simulink model "RRTMS_System_Architecture"  (R2026a)
settings: Solver=VariableStepAuto
settings Model: Creator=HP  LastModifiedBy=HP

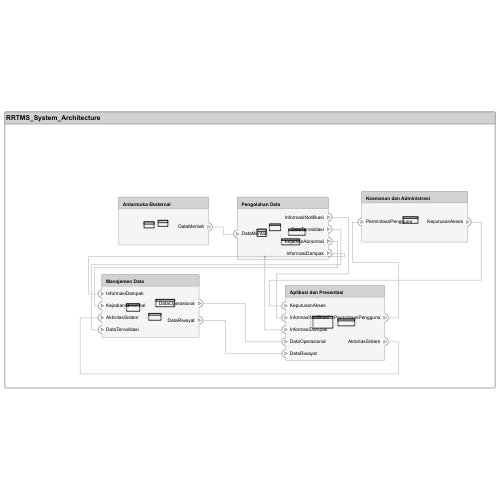
[thumbnail: Simulink's stored preview of the top-level diagram]
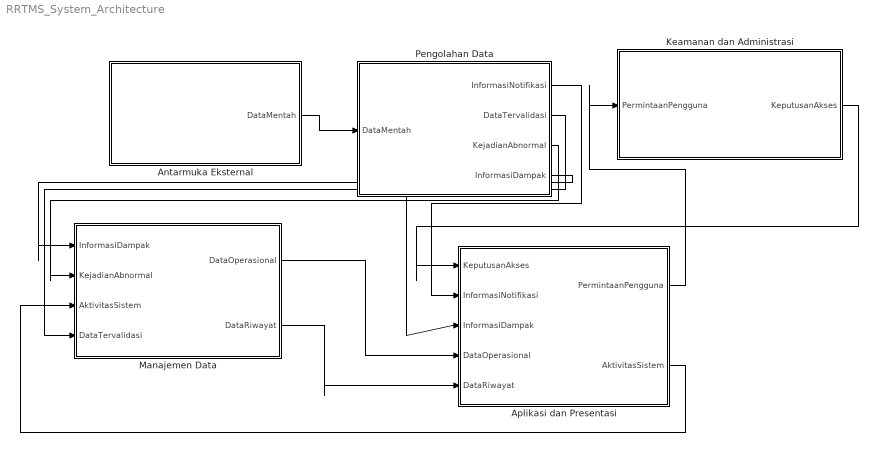
== system RRTMS_System_Architecture ==
  Antarmuka Eksternal : Subsystem
      settings: PortSchema="{\"entries\":[{\"content\":{\"headerSize\":26,\"margin\":15,\"minimumSpacing\":25,\"sides\":[{\"content\":{},\"type\":\"ConnectorPlacement.EquallySpacedRectSide\",\"uuid\":\"71f00674-931b-470b-b0fd-a692bb3b3063\"},{\"content\":{\"connectorIds\":[\"Out1\"],\"side\":\"RIGHT\"},\"type\":\"ConnectorPlacement.EquallySpacedRectSide\",\"uuid\":\"86d6e0cc-71b2-4a9b-97f1-d24c94197c14\"},{\"content\":{\"side\":\"TOP\"},\"type\":\"ConnectorPlacement.EquallySpacedRectSide\",\"uuid\":\"2847748d-1182-42d4-93ed-9e0e7089bed0\"}]},\"type\":\"ConnectorPlacement.EquallySpacedConnector\",\"uuid\":\"b969c393-021a-4397-a00e-d7d17b1fb0f6\"}],\"packageUris\":[\"http://schema.mathworks.com/mf0/Connector/R2020b\"],\"version\":\"1.0\"}"
  Aplikasi dan Presentasi : Subsystem
      settings: PortSchema="{\"entries\":[{\"content\":{\"headerSize\":26,\"margin\":15,\"minimumSpacing\":25,\"sides\":[{\"content\":{\"connectorIds\":[\"In1\",\"In2\",\"In5\",\"In3\",\"In4\"]},\"type\":\"ConnectorPlacement.EquallySpacedRectSide\",\"uuid\":\"71f00674-931b-470b-b0fd-a692bb3b3063\"},{\"content\":{\"connectorIds\":[\"Out1\",\"Out2\"],\"side\":\"RIGHT\"},\"type\":\"ConnectorPlacement.EquallySpacedRectSide\",\"uuid\":\"86d6e0cc-71b2-4a9b-97f1-d24c94197c14\"},{\"content\":{\"side\":\"TOP\"},\"type\":\"ConnectorPlacement.EquallySpacedRectSide\",\"uuid\":\"2847748d-1182-42d4-93ed-9e0e7089bed0\"}]},\"type\":\"ConnectorPlacement.EquallySpacedConnector\",\"uuid\":\"b969c393-021a-4397-a00e-d7d17b1fb0f6\"}],\"packageUris\":[\"http://schema.mathworks.com/mf0/Connector/R2020b\"],\"version\":\"1.0\"}"
  Keamanan dan Administrasi : Subsystem
      settings: PortSchema="{\"entries\":[{\"content\":{\"headerSize\":26,\"margin\":15,\"minimumSpacing\":25,\"sides\":[{\"content\":{\"connectorIds\":[\"In1\"]},\"type\":\"ConnectorPlacement.EquallySpacedRectSide\",\"uuid\":\"71f00674-931b-470b-b0fd-a692bb3b3063\"},{\"content\":{\"connectorIds\":[\"Out1\"],\"side\":\"RIGHT\"},\"type\":\"ConnectorPlacement.EquallySpacedRectSide\",\"uuid\":\"86d6e0cc-71b2-4a9b-97f1-d24c94197c14\"},{\"content\":{\"side\":\"TOP\"},\"type\":\"ConnectorPlacement.EquallySpacedRectSide\",\"uuid\":\"2847748d-1182-42d4-93ed-9e0e7089bed0\"}]},\"type\":\"ConnectorPlacement.EquallySpacedConnector\",\"uuid\":\"b969c393-021a-4397-a00e-d7d17b1fb0f6\"}],\"packageUris\":[\"http://schema.mathworks.com/mf0/Connector/R2020b\"],\"version\":\"1.0\"}"
  Manajemen Data : Subsystem
      settings: PortSchema="{\"entries\":[{\"content\":{\"headerSize\":26,\"margin\":15,\"minimumSpacing\":25,\"sides\":[{\"content\":{\"connectorIds\":[\"In1\",\"In2\",\"In3\",\"In4\"]},\"type\":\"ConnectorPlacement.EquallySpacedRectSide\",\"uuid\":\"71f00674-931b-470b-b0fd-a692bb3b3063\"},{\"content\":{\"connectorIds\":[\"Out2\",\"Out1\"],\"side\":\"RIGHT\"},\"type\":\"ConnectorPlacement.EquallySpacedRectSide\",\"uuid\":\"86d6e0cc-71b2-4a9b-97f1-d24c94197c14\"},{\"content\":{\"side\":\"TOP\"},\"type\":\"ConnectorPlacement.EquallySpacedRectSide\",\"uuid\":\"2847748d-1182-42d4-93ed-9e0e7089bed0\"}]},\"type\":\"ConnectorPlacement.EquallySpacedConnector\",\"uuid\":\"b969c393-021a-4397-a00e-d7d17b1fb0f6\"}],\"packageUris\":[\"http://schema.mathworks.com/mf0/Connector/R2020b\"],\"version\":\"1.0\"}"
  Pengolahan Data : Subsystem
      settings: PortSchema="{\"entries\":[{\"content\":{\"headerSize\":26,\"margin\":15,\"minimumSpacing\":25,\"sides\":[{\"content\":{\"connectorIds\":[\"In1\"]},\"type\":\"ConnectorPlacement.EquallySpacedRectSide\",\"uuid\":\"71f00674-931b-470b-b0fd-a692bb3b3063\"},{\"content\":{\"connectorIds\":[\"Out1\",\"Out3\",\"Out4\",\"Out2\"],\"side\":\"RIGHT\"},\"type\":\"ConnectorPlacement.EquallySpacedRectSide\",\"uuid\":\"86d6e0cc-71b2-4a9b-97f1-d24c94197c14\"},{\"content\":{\"side\":\"TOP\"},\"type\":\"ConnectorPlacement.EquallySpacedRectSide\",\"uuid\":\"2847748d-1182-42d4-93ed-9e0e7089bed0\"}]},\"type\":\"ConnectorPlacement.EquallySpacedConnector\",\"uuid\":\"b969c393-021a-4397-a00e-d7d17b1fb0f6\"}],\"packageUris\":[\"http://schema.mathworks.com/mf0/Connector/R2020b\"],\"version\":\"1.0\"}"
  wires:
  Antarmuka Eksternal/1(DataMentah) -> Pengolahan Data/1(DataMentah)
  Pengolahan Data/3(DataTervalidasi) -> Manajemen Data/4(DataTervalidasi)
  Pengolahan Data/4(KejadianAbnormal) -> Manajemen Data/2(KejadianAbnormal)
  Pengolahan Data/2(InformasiDampak) -> Aplikasi dan Presentasi/5(InformasiDampak), Manajemen Data/1(InformasiDampak)
  Manajemen Data/2(DataOperasional) -> Aplikasi dan Presentasi/3(DataOperasional)
  Manajemen Data/1(DataRiwayat) -> Aplikasi dan Presentasi/4(DataRiwayat)
  Pengolahan Data/1(InformasiNotifikasi) -> Aplikasi dan Presentasi/2(InformasiNotifikasi)
  Aplikasi dan Presentasi/2(AktivitasSistem) -> Manajemen Data/3(AktivitasSistem)
  Aplikasi dan Presentasi/1(PermintaanPengguna) -> Keamanan dan Administrasi/1(PermintaanPengguna)
  Keamanan dan Administrasi/1(KeputusanAkses) -> Aplikasi dan Presentasi/1(KeputusanAkses)

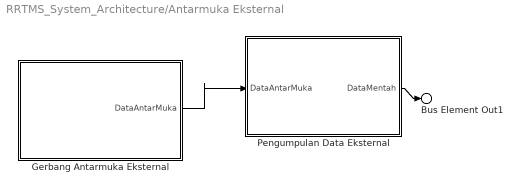
== system RRTMS_System_Architecture/Antarmuka Eksternal ==
  Gerbang Antarmuka Eksternal : Subsystem
      settings: PortSchema="{\"entries\":[{\"content\":{\"headerSize\":26,\"margin\":15,\"minimumSpacing\":25,\"sides\":[{\"content\":{},\"type\":\"ConnectorPlacement.EquallySpacedRectSide\",\"uuid\":\"71f00674-931b-470b-b0fd-a692bb3b3063\"},{\"content\":{\"connectorIds\":[\"Out1\"],\"side\":\"RIGHT\"},\"type\":\"ConnectorPlacement.EquallySpacedRectSide\",\"uuid\":\"86d6e0cc-71b2-4a9b-97f1-d24c94197c14\"},{\"content\":{\"side\":\"TOP\"},\"type\":\"ConnectorPlacement.EquallySpacedRectSide\",\"uuid\":\"2847748d-1182-42d4-93ed-9e0e7089bed0\"}]},\"type\":\"ConnectorPlacement.EquallySpacedConnector\",\"uuid\":\"b969c393-021a-4397-a00e-d7d17b1fb0f6\"}],\"packageUris\":[\"http://schema.mathworks.com/mf0/Connector/R2020b\"],\"version\":\"1.0\"}"
  Pengumpulan Data Eksternal : Subsystem
      settings: PortSchema="{\"entries\":[{\"content\":{\"headerSize\":26,\"margin\":15,\"minimumSpacing\":25,\"sides\":[{\"content\":{\"connectorIds\":[\"In1\"]},\"type\":\"ConnectorPlacement.EquallySpacedRectSide\",\"uuid\":\"71f00674-931b-470b-b0fd-a692bb3b3063\"},{\"content\":{\"connectorIds\":[\"Out1\"],\"side\":\"RIGHT\"},\"type\":\"ConnectorPlacement.EquallySpacedRectSide\",\"uuid\":\"86d6e0cc-71b2-4a9b-97f1-d24c94197c14\"},{\"content\":{\"side\":\"TOP\"},\"type\":\"ConnectorPlacement.EquallySpacedRectSide\",\"uuid\":\"2847748d-1182-42d4-93ed-9e0e7089bed0\"}]},\"type\":\"ConnectorPlacement.EquallySpacedConnector\",\"uuid\":\"b969c393-021a-4397-a00e-d7d17b1fb0f6\"}],\"packageUris\":[\"http://schema.mathworks.com/mf0/Connector/R2020b\"],\"version\":\"1.0\"}"
  Bus Element Out1 : Outport  PortName=DataMentah
  wires:
  Gerbang Antarmuka Eksternal/1(DataAntarMuka) -> Pengumpulan Data Eksternal/1(DataAntarMuka)
  Pengumpulan Data Eksternal/1(DataMentah) -> Bus Element Out1/1

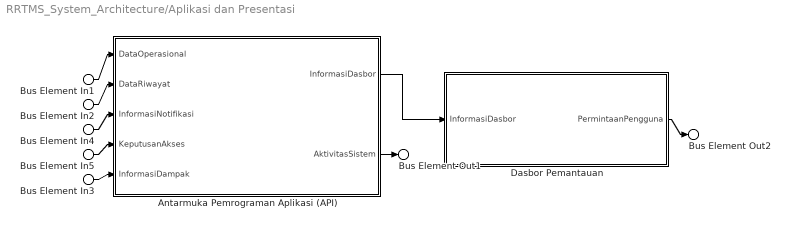
== system RRTMS_System_Architecture/Aplikasi dan Presentasi ==
  Bus Element In5 : Inport  PortName=KeputusanAkses
  Bus Element In4 : Inport  Port=2  PortName=InformasiNotifikasi
  Bus Element In1 : Inport  Port=3  PortName=DataOperasional
  Bus Element In2 : Inport  Port=4  PortName=DataRiwayat
  Bus Element In3 : Inport  Port=5  PortName=InformasiDampak
  Antarmuka Pemrograman Aplikasi (API) : Subsystem
      settings: PortSchema="{\"entries\":[{\"content\":{\"headerSize\":26,\"margin\":15,\"minimumSpacing\":25,\"sides\":[{\"content\":{\"connectorIds\":[\"In1\",\"In2\",\"In3\",\"In4\",\"In5\"]},\"type\":\"ConnectorPlacement.EquallySpacedRectSide\",\"uuid\":\"71f00674-931b-470b-b0fd-a692bb3b3063\"},{\"content\":{\"connectorIds\":[\"Out1\",\"Out2\"],\"side\":\"RIGHT\"},\"type\":\"ConnectorPlacement.EquallySpacedRectSide\",\"uuid\":\"86d6e0cc-71b2-4a9b-97f1-d24c94197c14\"},{\"content\":{\"side\":\"TOP\"},\"type\":\"ConnectorPlacement.EquallySpacedRectSide\",\"uuid\":\"2847748d-1182-42d4-93ed-9e0e7089bed0\"}]},\"type\":\"ConnectorPlacement.EquallySpacedConnector\",\"uuid\":\"b969c393-021a-4397-a00e-d7d17b1fb0f6\"}],\"packageUris\":[\"http://schema.mathworks.com/mf0/Connector/R2020b\"],\"version\":\"1.0\"}"
  Dasbor Pemantauan : Subsystem
      settings: PortSchema="{\"entries\":[{\"content\":{\"headerSize\":26,\"margin\":15,\"minimumSpacing\":25,\"sides\":[{\"content\":{\"connectorIds\":[\"In1\"]},\"type\":\"ConnectorPlacement.EquallySpacedRectSide\",\"uuid\":\"71f00674-931b-470b-b0fd-a692bb3b3063\"},{\"content\":{\"connectorIds\":[\"Out1\"],\"side\":\"RIGHT\"},\"type\":\"ConnectorPlacement.EquallySpacedRectSide\",\"uuid\":\"86d6e0cc-71b2-4a9b-97f1-d24c94197c14\"},{\"content\":{\"side\":\"TOP\"},\"type\":\"ConnectorPlacement.EquallySpacedRectSide\",\"uuid\":\"2847748d-1182-42d4-93ed-9e0e7089bed0\"}]},\"type\":\"ConnectorPlacement.EquallySpacedConnector\",\"uuid\":\"b969c393-021a-4397-a00e-d7d17b1fb0f6\"}],\"packageUris\":[\"http://schema.mathworks.com/mf0/Connector/R2020b\"],\"version\":\"1.0\"}"
  Bus Element Out2 : Outport  PortName=PermintaanPengguna
  Bus Element Out1 : Outport  Port=2  PortName=AktivitasSistem
  wires:
  Bus Element In1/1 -> Antarmuka Pemrograman Aplikasi (API)/1(DataOperasional)
  Bus Element In2/1 -> Antarmuka Pemrograman Aplikasi (API)/2(DataRiwayat)
  Bus Element In3/1 -> Antarmuka Pemrograman Aplikasi (API)/5(InformasiDampak)
  Bus Element In4/1 -> Antarmuka Pemrograman Aplikasi (API)/3(InformasiNotifikasi)
  Antarmuka Pemrograman Aplikasi (API)/1(InformasiDasbor) -> Dasbor Pemantauan/1(InformasiDasbor)
  Antarmuka Pemrograman Aplikasi (API)/2(AktivitasSistem) -> Bus Element Out1/1
  Dasbor Pemantauan/1(PermintaanPengguna) -> Bus Element Out2/1
  Bus Element In5/1 -> Antarmuka Pemrograman Aplikasi (API)/4(KeputusanAkses)

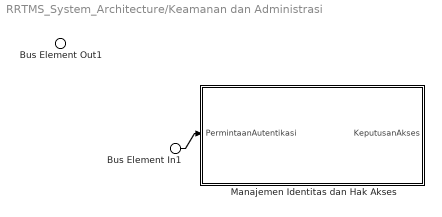
== system RRTMS_System_Architecture/Keamanan dan Administrasi ==
  Bus Element In1 : Inport  PortName=PermintaanPengguna
  Manajemen Identitas dan Hak Akses : Subsystem
      settings: PortSchema="{\"entries\":[{\"content\":{\"headerSize\":26,\"margin\":15,\"minimumSpacing\":25,\"sides\":[{\"content\":{\"connectorIds\":[\"In1\"]},\"type\":\"ConnectorPlacement.EquallySpacedRectSide\",\"uuid\":\"71f00674-931b-470b-b0fd-a692bb3b3063\"},{\"content\":{\"connectorIds\":[\"Out1\"],\"side\":\"RIGHT\"},\"type\":\"ConnectorPlacement.EquallySpacedRectSide\",\"uuid\":\"86d6e0cc-71b2-4a9b-97f1-d24c94197c14\"},{\"content\":{\"side\":\"TOP\"},\"type\":\"ConnectorPlacement.EquallySpacedRectSide\",\"uuid\":\"2847748d-1182-42d4-93ed-9e0e7089bed0\"}]},\"type\":\"ConnectorPlacement.EquallySpacedConnector\",\"uuid\":\"b969c393-021a-4397-a00e-d7d17b1fb0f6\"}],\"packageUris\":[\"http://schema.mathworks.com/mf0/Connector/R2020b\"],\"version\":\"1.0\"}"
  Bus Element Out1 : Outport  PortName=KeputusanAkses
  wires:
  Bus Element In1/1 -> Manajemen Identitas dan Hak Akses/1(PermintaanAutentikasi)

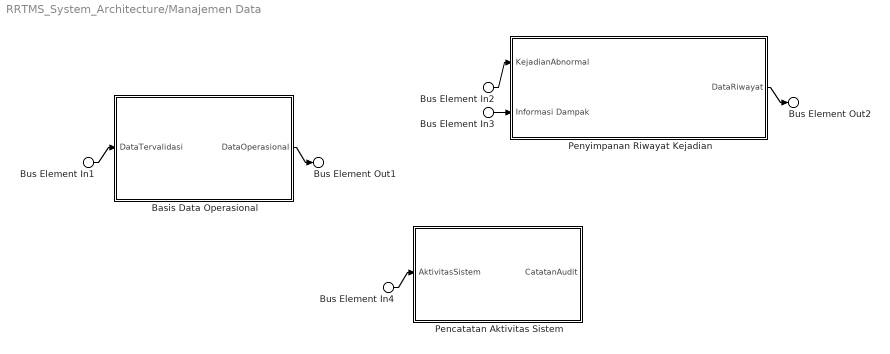
== system RRTMS_System_Architecture/Manajemen Data ==
  Bus Element In3 : Inport  PortName=InformasiDampak
  Bus Element In2 : Inport  Port=2  PortName=KejadianAbnormal
  Bus Element In4 : Inport  Port=3  PortName=AktivitasSistem
  Bus Element In1 : Inport  Port=4  PortName=DataTervalidasi
  Basis Data Operasional : Subsystem
      settings: PortSchema="{\"entries\":[{\"content\":{\"headerSize\":26,\"margin\":15,\"minimumSpacing\":25,\"sides\":[{\"content\":{\"connectorIds\":[\"In1\"]},\"type\":\"ConnectorPlacement.EquallySpacedRectSide\",\"uuid\":\"71f00674-931b-470b-b0fd-a692bb3b3063\"},{\"content\":{\"connectorIds\":[\"Out1\"],\"side\":\"RIGHT\"},\"type\":\"ConnectorPlacement.EquallySpacedRectSide\",\"uuid\":\"86d6e0cc-71b2-4a9b-97f1-d24c94197c14\"},{\"content\":{\"side\":\"TOP\"},\"type\":\"ConnectorPlacement.EquallySpacedRectSide\",\"uuid\":\"2847748d-1182-42d4-93ed-9e0e7089bed0\"}]},\"type\":\"ConnectorPlacement.EquallySpacedConnector\",\"uuid\":\"b969c393-021a-4397-a00e-d7d17b1fb0f6\"}],\"packageUris\":[\"http://schema.mathworks.com/mf0/Connector/R2020b\"],\"version\":\"1.0\"}"
  "Pencatatan Aktivitas Sistem " : Subsystem
      settings: PortSchema="{\"entries\":[{\"content\":{\"headerSize\":26,\"margin\":15,\"minimumSpacing\":25,\"sides\":[{\"content\":{\"connectorIds\":[\"In1\"]},\"type\":\"ConnectorPlacement.EquallySpacedRectSide\",\"uuid\":\"71f00674-931b-470b-b0fd-a692bb3b3063\"},{\"content\":{\"connectorIds\":[\"Out1\"],\"side\":\"RIGHT\"},\"type\":\"ConnectorPlacement.EquallySpacedRectSide\",\"uuid\":\"86d6e0cc-71b2-4a9b-97f1-d24c94197c14\"},{\"content\":{\"side\":\"TOP\"},\"type\":\"ConnectorPlacement.EquallySpacedRectSide\",\"uuid\":\"2847748d-1182-42d4-93ed-9e0e7089bed0\"}]},\"type\":\"ConnectorPlacement.EquallySpacedConnector\",\"uuid\":\"b969c393-021a-4397-a00e-d7d17b1fb0f6\"}],\"packageUris\":[\"http://schema.mathworks.com/mf0/Connector/R2020b\"],\"version\":\"1.0\"}"
  Penyimpanan Riwayat Kejadian : Subsystem
      settings: PortSchema="{\"entries\":[{\"content\":{\"headerSize\":26,\"margin\":15,\"minimumSpacing\":25,\"sides\":[{\"content\":{\"connectorIds\":[\"In1\",\"In2\"]},\"type\":\"ConnectorPlacement.EquallySpacedRectSide\",\"uuid\":\"71f00674-931b-470b-b0fd-a692bb3b3063\"},{\"content\":{\"connectorIds\":[\"Out1\"],\"side\":\"RIGHT\"},\"type\":\"ConnectorPlacement.EquallySpacedRectSide\",\"uuid\":\"86d6e0cc-71b2-4a9b-97f1-d24c94197c14\"},{\"content\":{\"side\":\"TOP\"},\"type\":\"ConnectorPlacement.EquallySpacedRectSide\",\"uuid\":\"2847748d-1182-42d4-93ed-9e0e7089bed0\"}]},\"type\":\"ConnectorPlacement.EquallySpacedConnector\",\"uuid\":\"b969c393-021a-4397-a00e-d7d17b1fb0f6\"}],\"packageUris\":[\"http://schema.mathworks.com/mf0/Connector/R2020b\"],\"version\":\"1.0\"}"
  Bus Element Out2 : Outport  PortName=DataRiwayat
  Bus Element Out1 : Outport  Port=2  PortName=DataOperasional
  wires:
  Bus Element In1/1 -> Basis Data Operasional/1(DataTervalidasi)
  Bus Element In2/1 -> Penyimpanan Riwayat Kejadian/1(KejadianAbnormal)
  Bus Element In3/1 -> Penyimpanan Riwayat Kejadian/2(Informasi Dampak)
  Basis Data Operasional/1(DataOperasional) -> Bus Element Out1/1
  Penyimpanan Riwayat Kejadian/1(DataRiwayat) -> Bus Element Out2/1
  Bus Element In4/1 -> "Pencatatan Aktivitas Sistem "/1(AktivitasSistem)

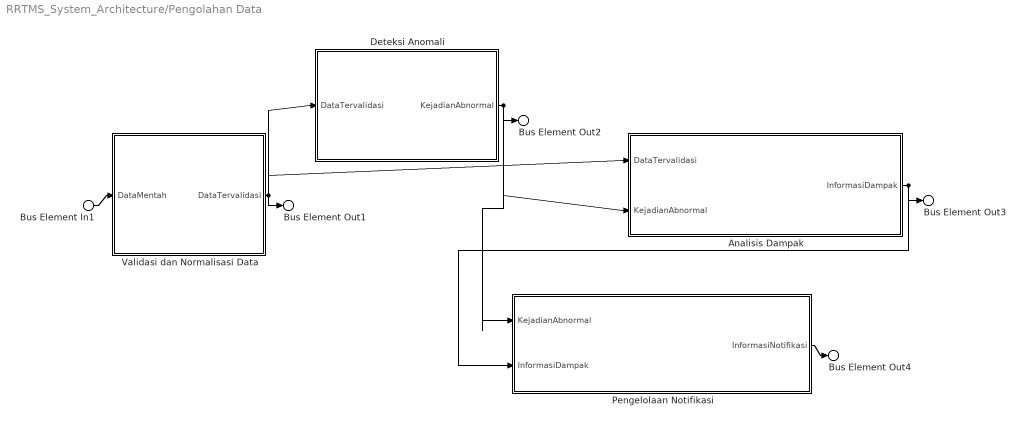
== system RRTMS_System_Architecture/Pengolahan Data ==
  Bus Element In1 : Inport  PortName=DataMentah
  Analisis Dampak : Subsystem
      settings: PortSchema="{\"entries\":[{\"content\":{\"headerSize\":26,\"margin\":15,\"minimumSpacing\":25,\"sides\":[{\"content\":{\"connectorIds\":[\"In1\",\"In2\"]},\"type\":\"ConnectorPlacement.EquallySpacedRectSide\",\"uuid\":\"71f00674-931b-470b-b0fd-a692bb3b3063\"},{\"content\":{\"connectorIds\":[\"Out1\"],\"side\":\"RIGHT\"},\"type\":\"ConnectorPlacement.EquallySpacedRectSide\",\"uuid\":\"86d6e0cc-71b2-4a9b-97f1-d24c94197c14\"},{\"content\":{\"side\":\"TOP\"},\"type\":\"ConnectorPlacement.EquallySpacedRectSide\",\"uuid\":\"2847748d-1182-42d4-93ed-9e0e7089bed0\"}]},\"type\":\"ConnectorPlacement.EquallySpacedConnector\",\"uuid\":\"b969c393-021a-4397-a00e-d7d17b1fb0f6\"}],\"packageUris\":[\"http://schema.mathworks.com/mf0/Connector/R2020b\"],\"version\":\"1.0\"}"
  Deteksi Anomali : Subsystem
      settings: PortSchema="{\"entries\":[{\"content\":{\"headerSize\":26,\"margin\":15,\"minimumSpacing\":25,\"sides\":[{\"content\":{\"connectorIds\":[\"In1\"]},\"type\":\"ConnectorPlacement.EquallySpacedRectSide\",\"uuid\":\"71f00674-931b-470b-b0fd-a692bb3b3063\"},{\"content\":{\"connectorIds\":[\"Out1\"],\"side\":\"RIGHT\"},\"type\":\"ConnectorPlacement.EquallySpacedRectSide\",\"uuid\":\"86d6e0cc-71b2-4a9b-97f1-d24c94197c14\"},{\"content\":{\"side\":\"TOP\"},\"type\":\"ConnectorPlacement.EquallySpacedRectSide\",\"uuid\":\"2847748d-1182-42d4-93ed-9e0e7089bed0\"}]},\"type\":\"ConnectorPlacement.EquallySpacedConnector\",\"uuid\":\"b969c393-021a-4397-a00e-d7d17b1fb0f6\"}],\"packageUris\":[\"http://schema.mathworks.com/mf0/Connector/R2020b\"],\"version\":\"1.0\"}"
  Pengelolaan Notifikasi : Subsystem
      settings: PortSchema="{\"entries\":[{\"content\":{\"headerSize\":26,\"margin\":15,\"minimumSpacing\":25,\"sides\":[{\"content\":{\"connectorIds\":[\"In1\",\"In2\"]},\"type\":\"ConnectorPlacement.EquallySpacedRectSide\",\"uuid\":\"71f00674-931b-470b-b0fd-a692bb3b3063\"},{\"content\":{\"connectorIds\":[\"Out1\"],\"side\":\"RIGHT\"},\"type\":\"ConnectorPlacement.EquallySpacedRectSide\",\"uuid\":\"86d6e0cc-71b2-4a9b-97f1-d24c94197c14\"},{\"content\":{\"side\":\"TOP\"},\"type\":\"ConnectorPlacement.EquallySpacedRectSide\",\"uuid\":\"2847748d-1182-42d4-93ed-9e0e7089bed0\"}]},\"type\":\"ConnectorPlacement.EquallySpacedConnector\",\"uuid\":\"b969c393-021a-4397-a00e-d7d17b1fb0f6\"}],\"packageUris\":[\"http://schema.mathworks.com/mf0/Connector/R2020b\"],\"version\":\"1.0\"}"
  Validasi dan Normalisasi Data : Subsystem
      settings: PortSchema="{\"entries\":[{\"content\":{\"headerSize\":26,\"margin\":15,\"minimumSpacing\":25,\"sides\":[{\"content\":{\"connectorIds\":[\"In1\"]},\"type\":\"ConnectorPlacement.EquallySpacedRectSide\",\"uuid\":\"71f00674-931b-470b-b0fd-a692bb3b3063\"},{\"content\":{\"connectorIds\":[\"Out1\"],\"side\":\"RIGHT\"},\"type\":\"ConnectorPlacement.EquallySpacedRectSide\",\"uuid\":\"86d6e0cc-71b2-4a9b-97f1-d24c94197c14\"},{\"content\":{\"side\":\"TOP\"},\"type\":\"ConnectorPlacement.EquallySpacedRectSide\",\"uuid\":\"2847748d-1182-42d4-93ed-9e0e7089bed0\"}]},\"type\":\"ConnectorPlacement.EquallySpacedConnector\",\"uuid\":\"b969c393-021a-4397-a00e-d7d17b1fb0f6\"}],\"packageUris\":[\"http://schema.mathworks.com/mf0/Connector/R2020b\"],\"version\":\"1.0\"}"
  Bus Element Out4 : Outport  PortName=InformasiNotifikasi
  Bus Element Out3 : Outport  Port=2  PortName=InformasiDampak
  Bus Element Out1 : Outport  Port=3  PortName=DataTervalidasi
  Bus Element Out2 : Outport  Port=4  PortName=KejadianAbnormal
  wires:
  Bus Element In1/1 -> Validasi dan Normalisasi Data/1(DataMentah)
  Validasi dan Normalisasi Data/1(DataTervalidasi) -> Deteksi Anomali/1(DataTervalidasi), Analisis Dampak/1(DataTervalidasi), Bus Element Out1/1
  Deteksi Anomali/1(KejadianAbnormal) -> Pengelolaan Notifikasi/1(KejadianAbnormal), Analisis Dampak/2(KejadianAbnormal), Bus Element Out2/1
  Analisis Dampak/1(InformasiDampak) -> Bus Element Out3/1, Pengelolaan Notifikasi/2(InformasiDampak)
  Pengelolaan Notifikasi/1(InformasiNotifikasi) -> Bus Element Out4/1

== system RRTMS_System_Architecture/Antarmuka Eksternal/Gerbang Antarmuka Eksternal ==
  Bus Element Out1 : Outport  PortName=DataAntarMuka

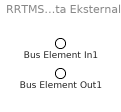
== system RRTMS_System_Architecture/Antarmuka Eksternal/Pengumpulan Data Eksternal ==
  Bus Element In1 : Inport  PortName=DataAntarMuka
  Bus Element Out1 : Outport  PortName=DataMentah

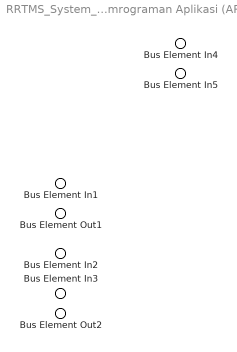
== system RRTMS_System_Architecture/Aplikasi dan Presentasi/Antarmuka Pemrograman Aplikasi (API) ==
  Bus Element In1 : Inport  PortName=DataOperasional
  Bus Element In2 : Inport  Port=2  PortName=DataRiwayat
  Bus Element In4 : Inport  Port=3  PortName=InformasiNotifikasi
  Bus Element In5 : Inport  Port=4  PortName=KeputusanAkses
  Bus Element In3 : Inport  Port=5  PortName=InformasiDampak
  Bus Element Out1 : Outport  PortName=InformasiDasbor
  Bus Element Out2 : Outport  Port=2  PortName=AktivitasSistem

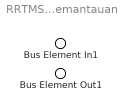
== system RRTMS_System_Architecture/Aplikasi dan Presentasi/Dasbor Pemantauan ==
  Bus Element In1 : Inport  PortName=InformasiDasbor
  Bus Element Out1 : Outport  PortName=PermintaanPengguna

== system RRTMS_System_Architecture/Keamanan dan Administrasi/Manajemen Identitas dan Hak Akses ==
  Bus Element In1 : Inport  PortName=PermintaanAutentikasi
  Bus Element Out1 : Outport  PortName=KeputusanAkses

== system RRTMS_System_Architecture/Manajemen Data/Basis Data Operasional ==
  Bus Element In1 : Inport  PortName=DataTervalidasi
  Bus Element Out1 : Outport  PortName=DataOperasional

== system RRTMS_System_Architecture/Manajemen Data/Pencatatan Aktivitas Sistem  ==
  Bus Element In1 : Inport  PortName=AktivitasSistem
  Bus Element Out1 : Outport  PortName=CatatanAudit

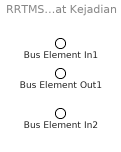
== system RRTMS_System_Architecture/Manajemen Data/Penyimpanan Riwayat Kejadian ==
  Bus Element In1 : Inport  PortName=KejadianAbnormal
  Bus Element In2 : Inport  Port=2  PortName=Informasi Dampak
  Bus Element Out1 : Outport  PortName=DataRiwayat

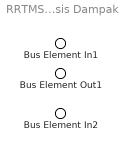
== system RRTMS_System_Architecture/Pengolahan Data/Analisis Dampak ==
  Bus Element In1 : Inport  PortName=DataTervalidasi
  Bus Element In2 : Inport  Port=2  PortName=KejadianAbnormal
  Bus Element Out1 : Outport  PortName=InformasiDampak

== system RRTMS_System_Architecture/Pengolahan Data/Deteksi Anomali ==
  Bus Element In1 : Inport  PortName=DataTervalidasi
  Bus Element Out1 : Outport  PortName=KejadianAbnormal

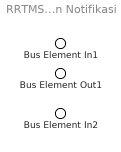
== system RRTMS_System_Architecture/Pengolahan Data/Pengelolaan Notifikasi ==
  Bus Element In1 : Inport  PortName=KejadianAbnormal
  Bus Element In2 : Inport  Port=2  PortName=InformasiDampak
  Bus Element Out1 : Outport  PortName=InformasiNotifikasi

== system RRTMS_System_Architecture/Pengolahan Data/Validasi dan Normalisasi Data ==
  Bus Element In1 : Inport  PortName=DataMentah
  Bus Element Out1 : Outport  PortName=DataTervalidasi
